simulink model "sphereVarMass"  (R2025a)
settings: Solver=ode4  StartTime=0  StopTime=900  FixedStep=0.01  MaxStep=0.01  RelTol=1e-3  EnableMultiTasking=on
values from neighbouring files (symbols this model uses):
  simu = simulationClass()    [wecSimInputFile.m]
  waves = waveClass('regular')    [wecSimInputFile.m]
undefined symbols (not defined in the file or in its folder): body, pto, X, Y, Z
libraries: nesl_utility x22, sm_lib x12, WECSim_Lib_Body_Elements x4, vrlib x1, matrix_library x1, WECSim_Lib_Frames x1, WECSim_Lib_PTOs x1
(part 4 of 4)

== matlab function sphereVarMass/Float/Hydrodynamic Body/Wave Radiation Forces Calculation/SS CI and Constant-Damping-CoeVariant Subsystem/Convolution Integral Calculation/Convolution Variant Subsystem/Convolution Integral Surface Calculation/convolutionIntegralSurface ==
  data: velocity input; timeExtrap output; hydroForceIndex input; hydroForceIndexInitial input; irkbSurfaceInput input; cicTime input; time input; FradExtrap output
function [timeExtrap, FradExtrap] = convolutionIntegralSurface(velocity, hydroForceIndex, hydroForceIndexInitial, irkbSurfaceInput, cicTime, time)

[timeExtrap, FradExtrap] = convolutionIntegralSurface(velocity, hydroForceIndex, hydroForceIndexInitial, irkbSurfaceInput, cicTime, time);

end

== matlab function sphereVarMass/Float/Hydrodynamic Body/Yaw Force Transforms/Yaw Force Transforms ==
  data: yaw input; F_Excitation output; dispGlobal input; F_RadiationDampingLocal input; F_AddedMassLocal input; F_ExcitationLocal input; F_RadiationDamping output; F_RestoringLocal input; F_AddedMass output; F_Restoring output
function [F_Excitation, F_RadiationDamping, F_AddedMass, F_Restoring] = fYawTransforms(yaw, dispGlobal, F_RadiationDampingLocal, F_AddedMassLocal, F_ExcitationLocal, F_RestoringLocal)

[F_Excitation, F_RadiationDamping, F_AddedMass, F_Restoring] = fYawTransforms(yaw, dispGlobal, F_RadiationDampingLocal, F_AddedMassLocal, F_ExcitationLocal, F_RestoringLocal);

end

== matlab function sphereVarMass/Float/Hydrodynamic Body/Yaw Kinematic Transforms/No B2B/Yaw Kinematic Transforms ==
  data: yaw input; dispLoc output; dispGlobal input; velGlobal input; accGlobal input; velLoc output; accLoc output
function [dispLoc, velLoc, accLoc] = kinYawTransform(yaw, dispGlobal, velGlobal, accGlobal)

[dispLoc, velLoc, accLoc] = kinYawTransformNoB2B(yaw, dispGlobal, velGlobal, accGlobal);

end

== matlab function sphereVarMass/Float/Hydrodynamic Body/Yaw Kinematic Transforms/With B2B/Yaw Kinematic Transforms ==
  data: yaw input; dispLoc output; dispGlobal input; velGlobal input; accGlobal input; velLoc output; accLoc output; numBody parameter
function [dispLoc, velLoc, accLoc] = kinYawTransformB2B(yaw, dispGlobal, velGlobal, accGlobal, numBody)

[dispLoc, velLoc, accLoc] = kinYawTransformB2B(yaw, dispGlobal, velGlobal, accGlobal, numBody);

end

== matlab function sphereVarMass/MATLAB Function ==
  data: time input; body1_hydroForceIndex output
function body1_hydroForceIndex = calcIndex(time)

body1_hydroForceIndex = calcIndex(time);

end

== matlab function sphereVarMass/Float/Hydrodynamic Body/Hydrostatic Restoring Force Calculation/Linear and Nonlinear Restoring Force Variant Subsystem/Nonlinear Hydrostatic Restoring Force/Restoring Forces ==
  data: x input; elv input; center input; f output; tnorm input; area input; rho input; g input; cg input; p output; mass input
function [f,p]  = nonLinearBuoyancy(x,elv,center,tnorm,area,rho,g,cg,mass)

[f,p]  = nonLinearBuoyancy(x,elv,center,tnorm,area,rho,g,cg,mass);

end

== matlab function sphereVarMass/Float/Hydrodynamic Body/Morison Element and Viscous Damping Force Calculation/Morison Element Variant Subsystem/Morison Element On/Irregular Wave Morison Force/MATLAB Function ==
  data: z input; f output; r input; Vel input; Accel input; Disp input; Area input; Cd input; Vol input; Ca input; Time input; rho input; waveDir input; waveSpread input; waterDepth input; k input; w input; A input; rampTime input; g input; randPhase input; dw input; currentSpeed input; currentDirection input; currentDepth input; currentOption input; simuMorison input
function f = irregWaveMorison(z,r,Vel,Accel,Disp,Area,Cd,Vol,Ca,Time,rho,waveDir,waveSpread,waterDepth,k,w,A,rampTime,g,randPhase,dw,currentSpeed,currentDirection,currentDepth,currentOption,simuMorison)

f = irregWaveMorison(z,r,Vel,Accel,Disp,Area,Cd,Vol,Ca,Time,rho,waveDir,waveSpread,waterDepth,k,w,A,rampTime,g,randPhase,dw,currentSpeed,currentDirection,currentDepth,currentOption,simuMorison);

end
